simulink model "gear_train"  (R2026a)
settings: Solver=VariableStepAuto
libraries: fl_lib x11, nesl_utility x6
settings Model: Creator=User  LastModifiedBy=User

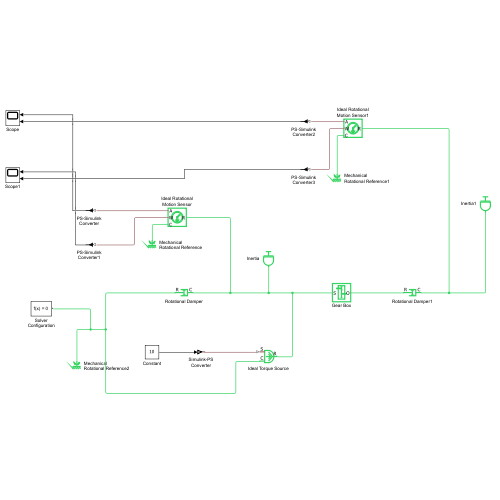
[thumbnail: Simulink's stored preview of the top-level diagram]
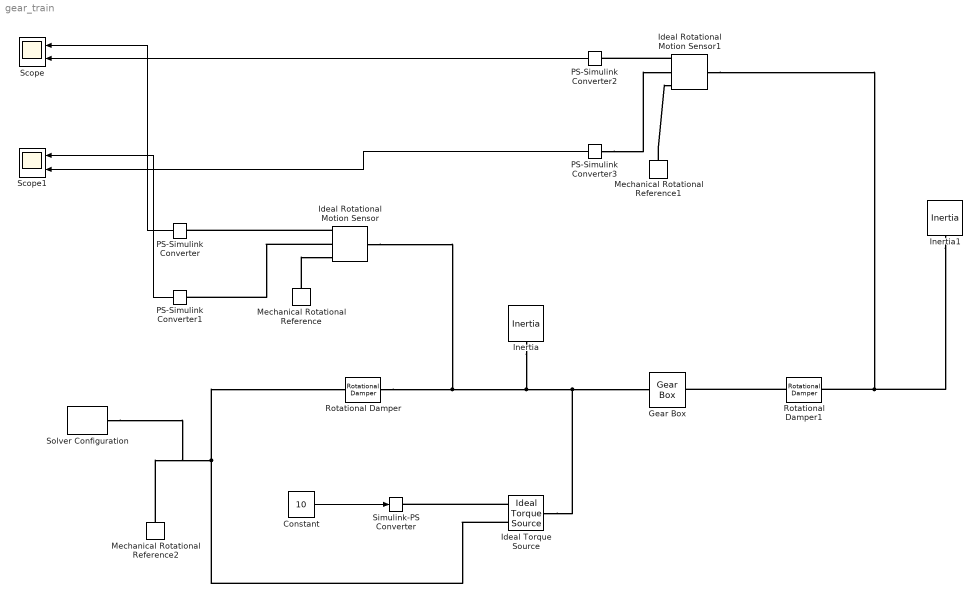
== system gear_train ==
  Constant : Constant  Value=10
  Gear Box : fl_lib/Mechanical/Mechanisms/Gear Box  ratio=40/100  t_in_specify=off  t_in_priority=None  t_in=0 N*m  t_in_nominal_specify=off  t_in_nominal_value=1  t_in_nominal_unit=N*m  t_out_specify=off  t_out_priority=None  t_out=0 N*m  t_out_nominal_specify=off  t_out_nominal_value=1  t_out_nominal_unit=N*m
  Ideal Rotational Motion Sensor : fl_lib/Mechanical/Mechanical Sensors/Ideal Rotational Motion Sensor  reference=foundation.enum.MeasurementReference.difference  acceleration_port=false  velocity_port=true  position_port=true  wrap_angle=false  offset=0 rad
  Ideal Rotational Motion Sensor1 : fl_lib/Mechanical/Mechanical Sensors/Ideal Rotational Motion Sensor  reference=foundation.enum.MeasurementReference.difference  acceleration_port=false  velocity_port=true  position_port=true  wrap_angle=false  offset=0 rad
  Ideal Torque Source : fl_lib/Mechanical/Mechanical Sources/Ideal Torque Source
  Inertia : fl_lib/Mechanical/Rotational Elements/Inertia  inertia=4.27e-07 kg*m^2  num_ports=foundation.enum.numPorts2.one  w_specify=off  w_priority=High  w=0 rad/s  w_nominal_specify=off  w_nominal_value=1  w_nominal_unit=rad/s  t_specify=off  t_priority=None  t=0 N*m  t_nominal_specify=off  t_nominal_value=1  t_nominal_unit=N*m
  Inertia1 : fl_lib/Mechanical/Rotational Elements/Inertia  inertia=1.0e-6 kg*m^2  num_ports=foundation.enum.numPorts2.one  w_specify=off  w_priority=High  w=0 rad/s  w_nominal_specify=off  w_nominal_value=1  w_nominal_unit=rad/s  t_specify=off  t_priority=None  t=0 N*m  t_nominal_specify=off  t_nominal_value=1  t_nominal_unit=N*m
  Mechanical Rotational Reference : fl_lib/Mechanical/Rotational Elements/Mechanical Rotational Reference
  Mechanical Rotational Reference1 : fl_lib/Mechanical/Rotational Elements/Mechanical Rotational Reference
  Mechanical Rotational Reference2 : fl_lib/Mechanical/Rotational Elements/Mechanical Rotational Reference
  PS-Simulink Converter{,1..3} (4 alike) : nesl_utility/PS-Simulink Converter  PhysicalDomain=network_engine_domain  SubClassName=ps_output  LeftPortType=input  RightPortType=output  PseudoPeriodic=off  Frequencies=[]  VectorFormat=inherit  Unit=inherit  AffineConversion=off
  Rotational Damper : fl_lib/Mechanical/Rotational Elements/Rotational Damper  D=0.0001 N*m*s/rad  w_specify=off  w_priority=None  w=0 rad/s  w_nominal_specify=off  w_nominal_value=1  w_nominal_unit=rad/s  t_specify=off  t_priority=None  t=0 N*m  t_nominal_specify=off  t_nominal_value=1  t_nominal_unit=N*m
  Rotational Damper1 : fl_lib/Mechanical/Rotational Elements/Rotational Damper  D=0.0001 N*m*s/rad  w_specify=off  w_priority=None  w=0 rad/s  w_nominal_specify=off  w_nominal_value=1  w_nominal_unit=rad/s  t_specify=off  t_priority=None  t=0 N*m  t_nominal_specify=off  t_nominal_value=1  t_nominal_unit=N*m
  Scope : Scope  NumInputPorts=2
      settings: ActiveDisplayYMinimum=-310100.93747269543  ActiveDisplayYMaximum=2.7909084372542594E+6
  Scope1 : Scope  NumInputPorts=2
      settings: ActiveDisplayYMinimum=46836.457532747736  ActiveDisplayYMaximum=224411.64159644739
  Simulink-PS Converter : nesl_utility/Simulink-PS Converter  PhysicalDomain=network_engine_domain  SubClassName=ps_input  LeftPortType=input  RightPortType=output  PseudoPeriodic=off  Frequencies=[]  NoiseDistribution=none  NoiseParameters=[]  Unit=1  AffineConversion=off  FilteringAndDerivatives=provide  SimscapeFilterOrder=1  InputFilterTimeConstant=0.001  UdotUserProvided=0
  Solver Configuration : nesl_utility/Solver Configuration  PhysicalDomain=network_engine_domain  SubClassName=solver  LeftPortType=input  RightPortType=generic  Tones=[]  Harmonics=[]  SimulateNoise=off  Profile=off  UseLocalSampling=off  EnableSwitchedLinearOptims=on  FrequencyDomain=off  UseCCode=off  RelTol=0.001  AbsTol=0.001  MinStep=1e-09  ToWorkspace=off  RevertToSquareIcSolve=off  NumHomotopyIterations=100  PhasorMode=off  PhasorModeNumHarmonics=1  ConsistencySolver=NEWTON_XTOL_AFTER_FTOL  CanonicalOrdering=CANONICAL  OptimizeIntermediates=OPTIMIZED  IndexReductionMethod=DerivativeReplacement  DoDC=off  ResidualTolerance=1e-09  ConsistencyTolSource=GLOBAL  ConsistencyAbsTol=0.001  ConsistencyRelTol=0.001  ConsistencyTolFactor=0.001  UseLocalSolver=off  LocalSolverChoice=NE_BACKWARD_EULER_ADVANCER  ResolveIndetEquations=on  FunctionEvalNumThread=1  LocalSolverSampleTime=0.001  DoFixedCost=off  MaxNonlinIter=3  MaxModeIter=2  ComputeImpulses=off  ImpulseIterations=2  LinearAlgebra=auto  LinearAlgebraNumThread=0  EquationFormulation=NE_TIME_EF  DelaysMemoryBudget=1024  AutomaticFiltering=on  FilteringTimeConstant=0.001  PartitionStorageMethod=AS_NEEDED  PartitionMemoryBudget=1024  PartitionMethod=ROBUST  MultibodyUseLocalSolver=off  MultibodyLocalSolverChoice=ODE1  MultibodyLocalSolverSampleTime=0.001
  wires:
  PS-Simulink Converter/1 -> Scope/1
  PS-Simulink Converter1/1 -> Scope1/1
  PS-Simulink Converter2/1 -> Scope/2
  PS-Simulink Converter3/1 -> Scope1/2
  Constant/1 -> Simulink-PS Converter/1
  connections:
  Ideal Rotational Motion Sensor/RConn3 -- PS-Simulink Converter/LConn1
  Ideal Rotational Motion Sensor/RConn2 -- PS-Simulink Converter1/LConn1
  Mechanical Rotational Reference/LConn1 -- Ideal Rotational Motion Sensor/RConn1
  Ideal Rotational Motion Sensor1/RConn3 -- PS-Simulink Converter2/LConn1
  PS-Simulink Converter3/LConn1 -- Ideal Rotational Motion Sensor1/RConn2
  Mechanical Rotational Reference1/LConn1 -- Ideal Rotational Motion Sensor1/RConn1
  Rotational Damper/RConn1 -- Ideal Rotational Motion Sensor/LConn1 -- Inertia/LConn1 -- Ideal Torque Source/LConn1 -- Gear Box/LConn1
  Rotational Damper1/LConn1 -- Gear Box/RConn1
  Inertia1/LConn1 -- Ideal Rotational Motion Sensor1/LConn1 -- Rotational Damper1/RConn1
  Ideal Torque Source/RConn1 -- Simulink-PS Converter/RConn1
  Ideal Torque Source/RConn2 -- Mechanical Rotational Reference2/LConn1 -- Solver Configuration/RConn1 -- Rotational Damper/LConn1
